simulink model "Ecualizador"  (R2026b)
settings: Solver=VariableStepAuto  StopTime=300
libraries: dspfdesign x15, dspsnks4 x1, dspvision x1
settings Model: Creator=USER  LastModifiedBy=huall
settings RTWCC: GPUComputeCapability=5.0

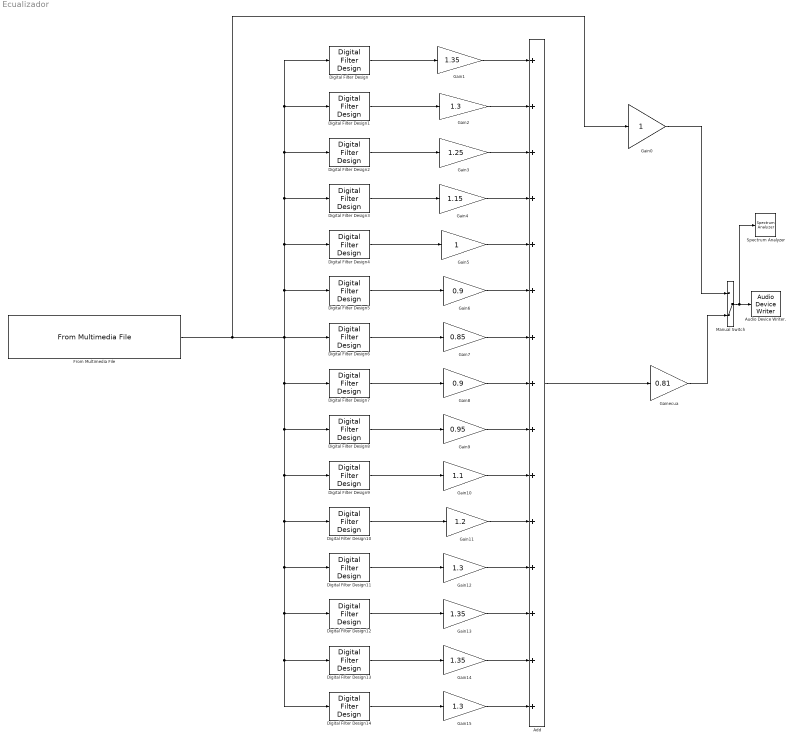
== system Ecualizador ==
  Add : Sum  Inputs=+++++++++++++++
  Audio Device Writer. : dspsnks4/Audio Device Writer  Driver=DirectSound  Device=Default  InheritSampleRate=on  SampleRate=44100  BitDepth=16-bit integer  BufferSize=4096  NumBuffers=10  DefaultOutputChannelMapping=on  OutputChannelMapping=1:2  OutputNumUnderrunSamples=off  DriverIdx=1  DeviceWarnFlag=''
  Digital Filter Design{,1..14} (15 alike) : dspfdesign/Digital Filter Design  mwdsp_browser_bugfix_var=off
  From Multimedia File : dspvision/From Multimedia File  inputFilename=C:\Users\huall\Downloads\E}cualizaodorLaptopAntigua\ECUALIZADOR\twenty one pilots - Ride (Official Video) - (256 Kbps).mp3  readRange=[5315332 Inf]  loop=on  numPlays=inf  outputStreams=Audio only  videoDataType=single  audioDataType=double  inheritSampleTime=on  userDefinedSampleTime=1/30  noAudioOutput=off  isIntensityVideo=off  fourcc=RGB  colorVideoFormat=Separate color signals  outputEOF=off  dataOrg=Column-major  audioFrameSize=1024  computeAudioFrameSize=off  outSamplingMode=Sample based
      settings: LibrarySourceBlock=audiosources/From Multimedia File
  Gain0 : Gain
  Gain1 : Gain  Gain=1.35
  Gain10 : Gain  Gain=1.1
  Gain11 : Gain  Gain=1.2
  Gain12 : Gain  Gain=1.3
  Gain13 : Gain  Gain=1.35
  Gain14 : Gain  Gain=1.35
  Gain15 : Gain  Gain=1.3
  Gain2 : Gain  Gain=1.3
  Gain3 : Gain  Gain=1.25
  Gain4 : Gain  Gain=1.15
  Gain5 : Gain
  Gain6 : Gain  Gain=0.9
  Gain7 : Gain  Gain=0.85
  Gain8 : Gain  Gain=0.9
  Gain9 : Gain  Gain=0.95
  Gainecua : Gain  Gain=0.81
  Manual Switch : ManualSwitch  CurrentSetting=0
  Spectrum Analyzer : SpectrumAnalyzer  WindowPosition=[1.000000,41.000000,1366.000000,705.000000,]  Visible=on  ScopeFrameLocation=window  Method=Welch  PlotAsTwoSidedSpectrum=off  FrequencyScale=Log  AveragingMethod=Exponential  ReferenceLoad=50  YLimits=[-143.6224 7.0183]  SelectedToolstripTab=spectrumAnalyzerToolstrip.spectrumTab
  wires:
  Manual Switch/1 -> Spectrum Analyzer/1, Audio Device Writer./1
  Add/1 -> Gainecua/1
  Gainecua/1 -> Manual Switch/2
  Gain0/1 -> Manual Switch/1
  Digital Filter Design1/1 -> Gain2/1
  Gain5/1 -> Add/5
  Gain2/1 -> Add/2
  Gain6/1 -> Add/6
  Digital Filter Design5/1 -> Gain6/1
  Digital Filter Design3/1 -> Gain4/1
  Digital Filter Design2/1 -> Gain3/1
  Gain3/1 -> Add/3
  Gain1/1 -> Add/1
  Gain4/1 -> Add/4
  Digital Filter Design/1 -> Gain1/1
  From Multimedia File/1 -> Gain0/1, Digital Filter Design/1, Digital Filter Design1/1, Digital Filter Design2/1, Digital Filter Design3/1, Digital Filter Design4/1, Digital Filter Design5/1, Digital Filter Design14/1, Digital Filter Design13/1, Digital Filter Design12/1, Digital Filter Design11/1, Digital Filter Design10/1, Digital Filter Design9/1, Digital Filter Design8/1, Digital Filter Design7/1, Digital Filter Design6/1
  Digital Filter Design4/1 -> Gain5/1
  Digital Filter Design6/1 -> Gain7/1
  Digital Filter Design7/1 -> Gain8/1
  Digital Filter Design8/1 -> Gain9/1
  Gain7/1 -> Add/7
  Gain8/1 -> Add/8
  Gain9/1 -> Add/9
  Digital Filter Design9/1 -> Gain10/1
  Digital Filter Design10/1 -> Gain11/1
  Digital Filter Design11/1 -> Gain12/1
  Gain12/1 -> Add/12
  Gain11/1 -> Add/11
  Gain10/1 -> Add/10
  Gain13/1 -> Add/13
  Gain15/1 -> Add/15
  Gain14/1 -> Add/14
  Digital Filter Design12/1 -> Gain13/1
  Digital Filter Design13/1 -> Gain14/1
  Digital Filter Design14/1 -> Gain15/1
